simulink model "P1_model_conventional"  (R2025b)
settings: Solver=ode4  StartTime=0.0  StopTime=4  FixedStep=20e-6  RelTol=1e-3
model workspace (MATLAB code in the model file):
  | % ---- 플랜트 (참값) ----
  | J  = 0.02;      % kg·m²
  | B  = 0.10;      % N·m·s  (참 감쇠)
  | 
  | % ---- 컨트롤러가 아는 값 ----
  | Bn   = 0.06;    % 공칭 감쇠 (−40%)
  | lam  = 30;      % rad/s
  | Ts   = 1e-3;    % 컨트롤러 주기 1 ms
  | umax = 6;       % 입력 한계 N·m  (진단 실행: 1e9)
  | 
  | % ---- 케이스 선택 ----
  | mode    = 1;    % 1: conventional, 2: transient-improved
  | zeta    = 0.3;  % 0.7 또는 0.3
  | wa      = 200;  % 200 또는 1000
  | sigma_n = 0;    % 0 또는 0.05
  | 
  | % ---- 유도되는 값 (자동 계산) ----
  | k_conv = J*lam^2/(4*zeta^2);
  | ka     = wa*Ts;
settings Model: Creator=Owner  LastModifiedBy=Owner

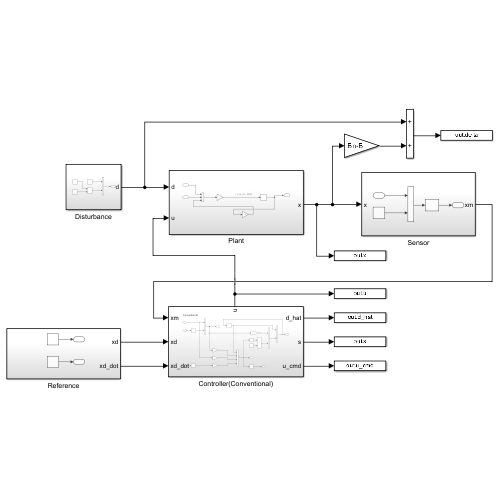
[thumbnail: Simulink's stored preview of the top-level diagram]
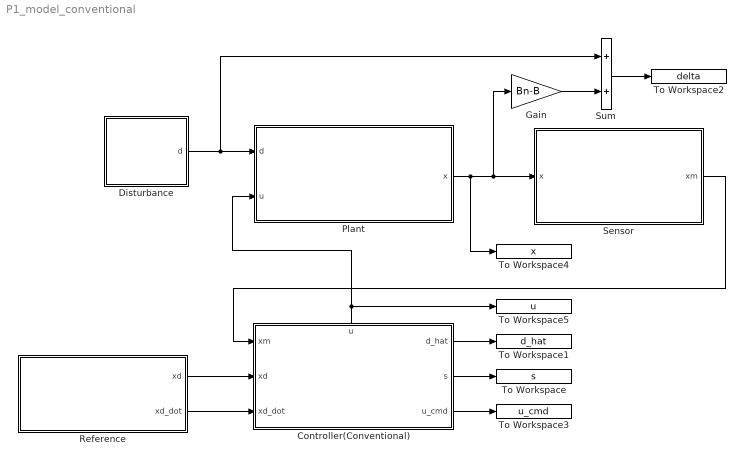
== system P1_model_conventional ==
  Controller(Conventional) : Subsystem
      settings: PortSchema="{\"entries\":[{\"content\":{\"sides\":[{\"content\":{\"connectorIds\":[\"In1\",\"In2\",\"In3\"]},\"type\":\"ConnectorPlacement.EquallySpacedRectSide\",\"uuid\":\"db018cbb-f712-44f0-9512-4d94f82516be\"},{\"content\":{\"connectorIds\":[\"Out1\",\"Out2\",\"Out3\"],\"side\":\"RIGHT\"},\"type\":\"ConnectorPlacement.EquallySpacedRectSide\",\"uuid\":\"79f58bb9-febf-4414-88b5-61586d37b576\"},{\"content\":{\"connectorIds\":[\"Out4\"],\"side\":\"TOP\"},\"type\":\"ConnectorPlacement.EquallySpacedRectSide\",\"uuid\":\"ac911475-5310-46a2-bcdf-979d5982e8b1\"}]},\"type\":\"ConnectorPlacement.EquallySpacedConnector\",\"uuid\":\"5be97a90-a621-4e93-a7ea-194a2e1030e6\"}],\"packageUris\":[\"http://schema.mathworks.com/mf0/Connector/R2020b\"],\"version\":\"1.0\"}"
  Disturbance : Subsystem
  Gain : Gain  Gain=Bn-B
  Plant : Subsystem
  Reference : Subsystem
  Sensor : Subsystem
  Sum : Sum
  To Workspace : ToWorkspace  VariableName=s  SaveFormat=Timeseries  SampleTime=-1
  To Workspace1 : ToWorkspace  VariableName=d_hat  SaveFormat=Timeseries  SampleTime=-1
  To Workspace2 : ToWorkspace  VariableName=delta  SaveFormat=Timeseries  SampleTime=-1
  To Workspace3 : ToWorkspace  VariableName=u_cmd  SaveFormat=Timeseries  SampleTime=-1
  To Workspace4 : ToWorkspace  VariableName=x  SaveFormat=Timeseries  SampleTime=-1
  To Workspace5 : ToWorkspace  VariableName=u  SaveFormat=Timeseries  SampleTime=-1
  wires:
  Disturbance/1(d) -> Sum/1, Plant/1(d)
  Plant/1(x) -> To Workspace4/1, Gain/1, Sensor/1(x)
  Sensor/1(xm) -> Controller(Conventional)/1(xm)
  Reference/1(xd) -> Controller(Conventional)/2(xd)
  Reference/2(xd_dot) -> Controller(Conventional)/3(xd_dot)
  Controller(Conventional)/4(u) -> Plant/2(u), To Workspace5/1
  Gain/1 -> Sum/2
  Controller(Conventional)/2(s) -> To Workspace/1
  Controller(Conventional)/1(d_hat) -> To Workspace1/1
  Controller(Conventional)/3(u_cmd) -> To Workspace3/1
  Sum/1 -> To Workspace2/1

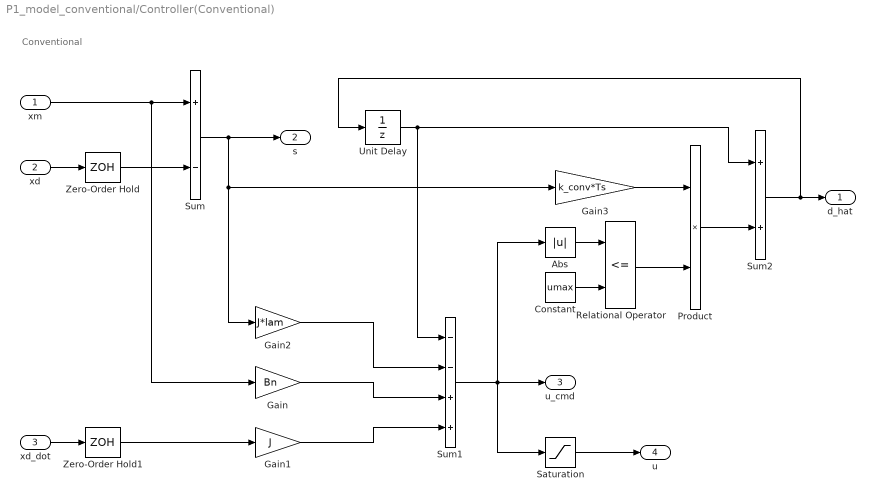
== system P1_model_conventional/Controller(Conventional) ==
  note: Conventional
  xm : Inport
  xd : Inport  Port=2
  xd_dot : Inport  Port=3
  Abs : Abs  SaturateOnIntegerOverflow=off
  Constant : Constant  Value=umax
  Gain : Gain  Gain=Bn
  Gain1 : Gain  Gain=J
  Gain2 : Gain  Gain=J*lam
  Gain3 : Gain  Gain=k_conv*Ts
  Product : Product
  Relational Operator : RelationalOperator  Operator=<=  OutDataTypeStr=boolean  RndMeth=Simplest  InputSameDT=off
  Saturation : Saturate  UpperLimit=umax  LowerLimit=-umax
  Sum : Sum  Inputs=+-
  Sum1 : Sum  Inputs=--++
  Sum2 : Sum
  Unit Delay : UnitDelay  SampleTime=Ts  HasFrameUpgradeWarning=on
  Zero-Order Hold : ZeroOrderHold  SampleTime=Ts
  Zero-Order Hold1 : ZeroOrderHold  SampleTime=Ts
  d_hat : Outport
  s : Outport  Port=2
  u_cmd : Outport  Port=3
  u : Outport  Port=4
  wires:
  xd/1 -> Zero-Order Hold/1
  xd_dot/1 -> Zero-Order Hold1/1
  Zero-Order Hold/1 -> Sum/2
  xm/1 -> Gain/1, Sum/1
  Sum/1 -> Gain3/1, Gain2/1, s/1
  Sum1/1 -> Abs/1, Saturation/1, u_cmd/1
  Zero-Order Hold1/1 -> Gain1/1
  Gain/1 -> Sum1/3
  Gain1/1 -> Sum1/4
  Saturation/1 -> u/1
  Gain2/1 -> Sum1/2
  Constant/1 -> Relational Operator/2
  Abs/1 -> Relational Operator/1
  Relational Operator/1 -> Product/2
  Gain3/1 -> Product/1
  Product/1 -> Sum2/2
  Sum2/1 -> Unit Delay/1, d_hat/1
  Unit Delay/1 -> Sum1/1, Sum2/1

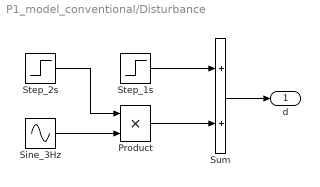
== system P1_model_conventional/Disturbance ==
  Product : Product
  Sine_3Hz : Sin  Amplitude=0.2  Frequency=6*pi  SampleTime=0
  Step_1s : Step  After=0.5  SampleTime=0
  Step_2s : Step  Time=2  SampleTime=0
  Sum : Sum
  d : Outport
  wires:
  Step_1s/1 -> Sum/1
  Product/1 -> Sum/2
  Step_2s/1 -> Product/1
  Sine_3Hz/1 -> Product/2
  Sum/1 -> d/1

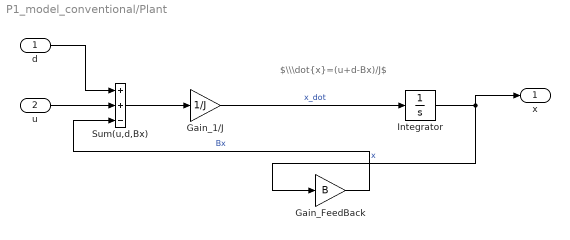
== system P1_model_conventional/Plant ==
  note: $\\\dot{x}=(u+d-Bx)/J$
  d : Inport
  u : Inport  Port=2
  Gain_1/J : Gain  Gain=1/J
  Gain_FeedBack : Gain  Gain=B
  Integrator : Integrator
  Sum(u,d,Bx) : Sum  Inputs=++-
  x : Outport
  wires:
  u/1 -> Sum(u,d,Bx)/2
  Sum(u,d,Bx)/1 -> Gain_1/J/1
  Gain_1/J/1 -> Integrator/1  "x_dot"
  Integrator/1 -> x/1, Gain_FeedBack/1  "x"
  Gain_FeedBack/1 -> Sum(u,d,Bx)/3  "Bx"
  d/1 -> Sum(u,d,Bx)/1

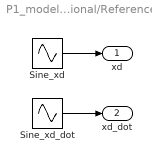
== system P1_model_conventional/Reference ==
  Sine_xd : Sin  Amplitude=40  Frequency=2*pi  SampleTime=0
  Sine_xd_dot : Sin  Amplitude=80*pi  Frequency=2*pi  Phase=pi/2  SampleTime=0
  xd : Outport
  xd_dot : Outport  Port=2
  wires:
  Sine_xd/1 -> xd/1
  Sine_xd_dot/1 -> xd_dot/1

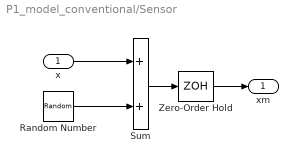
== system P1_model_conventional/Sensor ==
  x : Inport
  Random Number : RandomNumber  Variance=sigma_n^2  Seed=1  SampleTime=Ts
  Sum : Sum
  Zero-Order Hold : ZeroOrderHold  SampleTime=Ts
  xm : Outport
  wires:
  Random Number/1 -> Sum/2
  x/1 -> Sum/1
  Sum/1 -> Zero-Order Hold/1
  Zero-Order Hold/1 -> xm/1
